simulink model "Simulasi"  (R2020a)
settings: Solver=VariableStepAuto  StartTime=0.0  StopTime=10.0  RelTol=1e-3
settings Model: Creator=LENOVO  LastModifiedBy=LENOVO

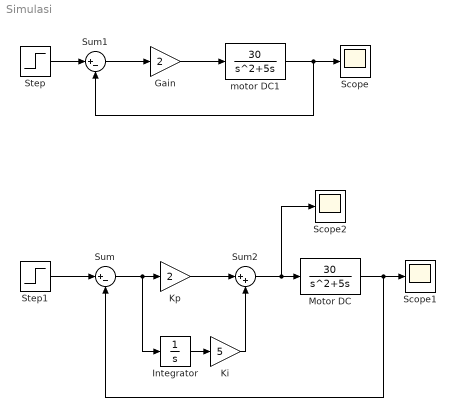
== system Simulasi ==
  Gain : Gain  Gain=2
  Integrator : Integrator
  Ki : Gain  Gain=5
  Kp : Gain  Gain=2
  Motor DC : TransferFcn  Numerator=[30]  Denominator=[1 5 0]
  Scope : Scope
  Scope1 : Scope
  Scope2 : Scope
  Step : Step  Time=0  SampleTime=0
  Step1 : Step  Time=0  SampleTime=0
  Sum : Sum  Inputs=|+-
  Sum1 : Sum  Inputs=|+-
  Sum2 : Sum  Inputs=|++
  motor DC1 : TransferFcn  Numerator=[30]  Denominator=[1 5 0]
  wires:
  Step/1 -> Sum1/1
  Gain/1 -> motor DC1/1
  Sum1/1 -> Gain/1
  motor DC1/1 -> Sum1/2, Scope/1
  Step1/1 -> Sum/1
  Kp/1 -> Sum2/1
  Sum2/1 -> Scope2/1, Motor DC/1
  Motor DC/1 -> Scope1/1, Sum/2
  Sum/1 -> Integrator/1, Kp/1
  Integrator/1 -> Ki/1
  Ki/1 -> Sum2/2
